simulink model "Wind_DFIG_Reused_R2"  (R2026a)
settings: Solver=ode15s  StopTime=DFIG.Simulation.StopTime  MaxStep=Base.Simulation.MaxStep
InitFcn:
  | root=fileparts(fileparts(get_param(bdroot,'FileName'))); run(fullfile(root,'parameters','init_wind_dfig_reused_r2.m'));
undefined symbols (not defined in the file): Base, Control, Converter, DFIG, Filter, Grid, Wind
libraries: nesl_utility x15, ee_lib x13, fl_lib x5, simulink x1
(part 2 of 2)

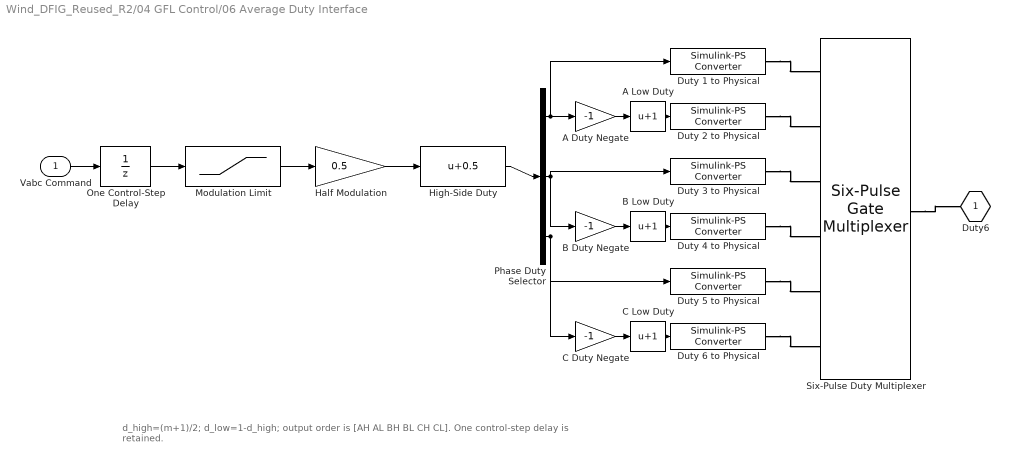
== system Wind_DFIG_Reused_R2/04 GFL Control/06 Average Duty Interface ==
  note: d_high=(m+1)/2; d_low=1-d_high; output order is [AH AL BH BL CH CL]. One control-step delay is retained.
  Vabc Command : Inport
  A Duty Negate : Gain  Gain=-1
  A Low Duty : Bias  Bias=1  SaturateOnIntegerOverflow=off
  B Duty Negate : Gain  Gain=-1
  B Low Duty : Bias  Bias=1  SaturateOnIntegerOverflow=off
  C Duty Negate : Gain  Gain=-1
  C Low Duty : Bias  Bias=1  SaturateOnIntegerOverflow=off
  Duty 1 to Physical : nesl_utility/Simulink-PS Converter  PhysicalDomain=network_engine_domain  SubClassName=ps_input  LeftPortType=input  RightPortType=output  PseudoPeriodic=off  Frequencies=[]  NoiseDistribution=none  NoiseParameters=[]  Unit=V  AffineConversion=off  FilteringAndDerivatives=provide  SimscapeFilterOrder=1  InputFilterTimeConstant=0.001  UdotUserProvided=0
  Duty 2 to Physical : nesl_utility/Simulink-PS Converter  PhysicalDomain=network_engine_domain  SubClassName=ps_input  LeftPortType=input  RightPortType=output  PseudoPeriodic=off  Frequencies=[]  NoiseDistribution=none  NoiseParameters=[]  Unit=V  AffineConversion=off  FilteringAndDerivatives=provide  SimscapeFilterOrder=1  InputFilterTimeConstant=0.001  UdotUserProvided=0
  Duty 3 to Physical : nesl_utility/Simulink-PS Converter  PhysicalDomain=network_engine_domain  SubClassName=ps_input  LeftPortType=input  RightPortType=output  PseudoPeriodic=off  Frequencies=[]  NoiseDistribution=none  NoiseParameters=[]  Unit=V  AffineConversion=off  FilteringAndDerivatives=provide  SimscapeFilterOrder=1  InputFilterTimeConstant=0.001  UdotUserProvided=0
  Duty 4 to Physical : nesl_utility/Simulink-PS Converter  PhysicalDomain=network_engine_domain  SubClassName=ps_input  LeftPortType=input  RightPortType=output  PseudoPeriodic=off  Frequencies=[]  NoiseDistribution=none  NoiseParameters=[]  Unit=V  AffineConversion=off  FilteringAndDerivatives=provide  SimscapeFilterOrder=1  InputFilterTimeConstant=0.001  UdotUserProvided=0
  Duty 5 to Physical : nesl_utility/Simulink-PS Converter  PhysicalDomain=network_engine_domain  SubClassName=ps_input  LeftPortType=input  RightPortType=output  PseudoPeriodic=off  Frequencies=[]  NoiseDistribution=none  NoiseParameters=[]  Unit=V  AffineConversion=off  FilteringAndDerivatives=provide  SimscapeFilterOrder=1  InputFilterTimeConstant=0.001  UdotUserProvided=0
  Duty 6 to Physical : nesl_utility/Simulink-PS Converter  PhysicalDomain=network_engine_domain  SubClassName=ps_input  LeftPortType=input  RightPortType=output  PseudoPeriodic=off  Frequencies=[]  NoiseDistribution=none  NoiseParameters=[]  Unit=V  AffineConversion=off  FilteringAndDerivatives=provide  SimscapeFilterOrder=1  InputFilterTimeConstant=0.001  UdotUserProvided=0
  Half Modulation : Gain  Gain=0.5
  High-Side Duty : Bias  Bias=0.5  SaturateOnIntegerOverflow=off
  Modulation Limit : Saturate  UpperLimit=Converter.ModulationMax  LowerLimit=-Converter.ModulationMax
  One Control-Step Delay : UnitDelay  InitialCondition=[0 0 0]  SampleTime=Control.Ts
  Phase Duty Selector : Demux  Outputs=3
  Six-Pulse Duty Multiplexer : ee_lib/Semiconductors & Converters/Converters/Six-Pulse Gate Multiplexer  port_option=ee.enum.controlport.ps
  Duty6 : PMIOPort  Side=Right
  wires:
  Vabc Command/1 -> One Control-Step Delay/1
  One Control-Step Delay/1 -> Modulation Limit/1
  Modulation Limit/1 -> Half Modulation/1
  Half Modulation/1 -> High-Side Duty/1
  High-Side Duty/1 -> Phase Duty Selector/1
  Phase Duty Selector/1 -> Duty 1 to Physical/1, A Duty Negate/1
  A Duty Negate/1 -> A Low Duty/1
  A Low Duty/1 -> Duty 2 to Physical/1
  Phase Duty Selector/2 -> Duty 3 to Physical/1, B Duty Negate/1
  B Duty Negate/1 -> B Low Duty/1
  B Low Duty/1 -> Duty 4 to Physical/1
  Phase Duty Selector/3 -> Duty 5 to Physical/1, C Duty Negate/1
  C Duty Negate/1 -> C Low Duty/1
  C Low Duty/1 -> Duty 6 to Physical/1
  connections:
  Duty 1 to Physical/RConn1 -- Six-Pulse Duty Multiplexer/LConn1
  Duty 2 to Physical/RConn1 -- Six-Pulse Duty Multiplexer/LConn2
  Duty 3 to Physical/RConn1 -- Six-Pulse Duty Multiplexer/LConn3
  Duty 4 to Physical/RConn1 -- Six-Pulse Duty Multiplexer/LConn4
  Duty 5 to Physical/RConn1 -- Six-Pulse Duty Multiplexer/LConn5
  Duty 6 to Physical/RConn1 -- Six-Pulse Duty Multiplexer/LConn6
  Six-Pulse Duty Multiplexer/RConn1 -- Duty6/RConn1

== system Wind_DFIG_Reused_R2/02 DFIG and Average RSC/02 Wound-Rotor DFIG dq Plant/01 Stator Voltage Equations ==
  Stator Current dq A : Inport
  Stator Flux dq Wb : Inport  Port=2
  Demux Is : Demux  Outputs=2
  Demux Psis : Demux  Outputs=2
  Demux Vs : Demux  Outputs=2
  Mux dPsi_s : Mux  Inputs=2
  Rs ids : Gain  Gain=DFIG.Machine.Rs
  Rs iqs : Gain  Gain=DFIG.Machine.Rs
  Stator Grid Voltage dq : Constant  Value=DFIG.Grid.Vdq
  d_psids_sum : Sum  Inputs=+-+
  d_psiqs_sum : Sum  Inputs=+--
  ws psids : Gain  Gain=DFIG.Base.ws
  ws psiqs : Gain  Gain=DFIG.Base.ws
  dPsi_sdq_dt : Outport
  wires:
  Stator Grid Voltage dq/1 -> Demux Vs/1
  Stator Current dq A/1 -> Demux Is/1
  Stator Flux dq Wb/1 -> Demux Psis/1
  Demux Is/1 -> Rs ids/1
  Demux Is/2 -> Rs iqs/1
  Demux Psis/1 -> ws psids/1
  Demux Psis/2 -> ws psiqs/1
  Demux Vs/1 -> d_psids_sum/1
  Rs ids/1 -> d_psids_sum/2
  ws psiqs/1 -> d_psids_sum/3
  Demux Vs/2 -> d_psiqs_sum/1
  Rs iqs/1 -> d_psiqs_sum/2
  ws psids/1 -> d_psiqs_sum/3
  d_psids_sum/1 -> Mux dPsi_s/1
  d_psiqs_sum/1 -> Mux dPsi_s/2
  Mux dPsi_s/1 -> dPsi_sdq_dt/1

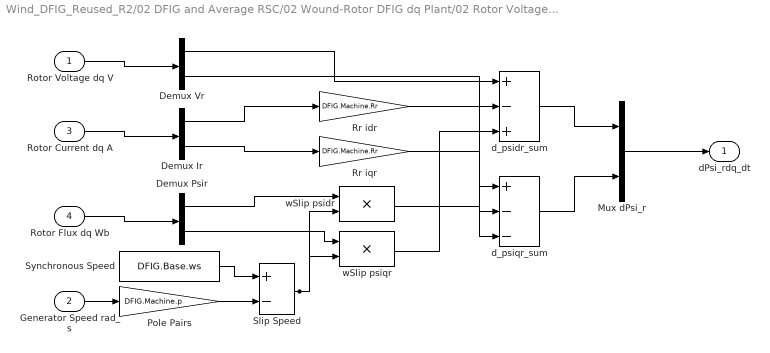
== system Wind_DFIG_Reused_R2/02 DFIG and Average RSC/02 Wound-Rotor DFIG dq Plant/02 Rotor Voltage Equations ==
  Rotor Voltage dq V : Inport
  Generator Speed rad_s : Inport  Port=2
  Rotor Current dq A : Inport  Port=3
  Rotor Flux dq Wb : Inport  Port=4
  Demux Ir : Demux  Outputs=2
  Demux Psir : Demux  Outputs=2
  Demux Vr : Demux  Outputs=2
  Mux dPsi_r : Mux  Inputs=2
  Pole Pairs : Gain  Gain=DFIG.Machine.p
  Rr idr : Gain  Gain=DFIG.Machine.Rr
  Rr iqr : Gain  Gain=DFIG.Machine.Rr
  Slip Speed : Sum  Inputs=+-
  Synchronous Speed : Constant  Value=DFIG.Base.ws
  d_psidr_sum : Sum  Inputs=+-+
  d_psiqr_sum : Sum  Inputs=+--
  wSlip psidr : Product  Inputs=**
  wSlip psiqr : Product  Inputs=**
  dPsi_rdq_dt : Outport
  wires:
  Rotor Voltage dq V/1 -> Demux Vr/1
  Rotor Current dq A/1 -> Demux Ir/1
  Rotor Flux dq Wb/1 -> Demux Psir/1
  Generator Speed rad_s/1 -> Pole Pairs/1
  Synchronous Speed/1 -> Slip Speed/1
  Pole Pairs/1 -> Slip Speed/2
  Demux Ir/1 -> Rr idr/1
  Demux Ir/2 -> Rr iqr/1
  Demux Psir/1 -> wSlip psidr/1
  Slip Speed/1 -> wSlip psidr/2, wSlip psiqr/2
  Demux Psir/2 -> wSlip psiqr/1
  Demux Vr/1 -> d_psidr_sum/1
  Rr idr/1 -> d_psidr_sum/2
  wSlip psiqr/1 -> d_psidr_sum/3
  Demux Vr/2 -> d_psiqr_sum/1
  Rr iqr/1 -> d_psiqr_sum/2
  wSlip psidr/1 -> d_psiqr_sum/3
  d_psidr_sum/1 -> Mux dPsi_r/1
  d_psiqr_sum/1 -> Mux dPsi_r/2
  Mux dPsi_r/1 -> dPsi_rdq_dt/1

== system Wind_DFIG_Reused_R2/02 DFIG and Average RSC/02 Wound-Rotor DFIG dq Plant/03 Flux Integrator and Inductance Matrix ==
  dPsi_sdq_dt : Inport
  dPsi_rdq_dt : Inport  Port=2
  Flux State Integrator : Integrator  InitialCondition=DFIG.Initial.flux
  Flux to Current Matrix : Gain  Gain=DFIG.Machine.CurrentFromFlux  Multiplication=Matrix(K*u)
  Mux State Derivative : Mux  Inputs=2
  Split Stator Rotor Current : Demux  Outputs=[2 2]
  Split Stator Rotor Flux : Demux  Outputs=[2 2]
  Stator Current dq A : Outport
  Rotor Current dq A : Outport  Port=2
  Stator Flux dq Wb : Outport  Port=3
  Rotor Flux dq Wb : Outport  Port=4
  wires:
  dPsi_sdq_dt/1 -> Mux State Derivative/1
  dPsi_rdq_dt/1 -> Mux State Derivative/2
  Mux State Derivative/1 -> Flux State Integrator/1
  Flux State Integrator/1 -> Flux to Current Matrix/1, Split Stator Rotor Flux/1
  Flux to Current Matrix/1 -> Split Stator Rotor Current/1
  Split Stator Rotor Current/1 -> Stator Current dq A/1
  Split Stator Rotor Current/2 -> Rotor Current dq A/1
  Split Stator Rotor Flux/1 -> Stator Flux dq Wb/1
  Split Stator Rotor Flux/2 -> Rotor Flux dq Wb/1

== system Wind_DFIG_Reused_R2/02 DFIG and Average RSC/02 Wound-Rotor DFIG dq Plant/04 Electromagnetic Torque ==
  Stator Current dq A : Inport
  Stator Flux dq Wb : Inport  Port=2
  Air-Gap Flux Cross Product : Sum  Inputs=+-
  Demux Is : Demux  Outputs=2
  Demux Psis : Demux  Outputs=2
  Torque Constant 1.5p : Gain  Gain=1.5*DFIG.Machine.p
  psids iqs : Product  Inputs=**
  psiqs ids : Product  Inputs=**
  Electromagnetic Torque Nm : Outport
  wires:
  Stator Current dq A/1 -> Demux Is/1
  Stator Flux dq Wb/1 -> Demux Psis/1
  Demux Psis/1 -> psids iqs/1
  Demux Is/2 -> psids iqs/2
  Demux Psis/2 -> psiqs ids/1
  Demux Is/1 -> psiqs ids/2
  psids iqs/1 -> Air-Gap Flux Cross Product/1
  psiqs ids/1 -> Air-Gap Flux Cross Product/2
  Air-Gap Flux Cross Product/1 -> Torque Constant 1.5p/1
  Torque Constant 1.5p/1 -> Electromagnetic Torque Nm/1

== system Wind_DFIG_Reused_R2/02 DFIG and Average RSC/03 Rotor-Side Average Converter Control/01 Stator-Flux Current Reference ==
  Torque Reference Nm : Inport
  Idr Magnetizing Reference : Constant  Value=DFIG.RSC.idrRef
  Torque to Iqr Gain : Gain  Gain=DFIG.RSC.torqueToIqr
  Idr_ref_raw_A : Outport
  Iqr_ref_raw_A : Outport  Port=2
  wires:
  Idr Magnetizing Reference/1 -> Idr_ref_raw_A/1
  Torque Reference Nm/1 -> Torque to Iqr Gain/1
  Torque to Iqr Gain/1 -> Iqr_ref_raw_A/1

== system Wind_DFIG_Reused_R2/02 DFIG and Average RSC/03 Rotor-Side Average Converter Control/02 Circular Rotor Current Limiter ==
  Idr_ref_raw_A : Inport
  Iqr_ref_raw_A : Inport  Port=2
  Circular Limit Scale : MinMax  Inputs=2
  Idr Limited : Product  Inputs=**
  Idr Squared : Math  Operator=square
  Iqr Limited : Product  Inputs=**
  Iqr Squared : Math  Operator=square
  Limit Ratio : Product  Inputs=*/
  Magnitude Floor : Constant
  Magnitude Squared : Sum
  Reference Magnitude : Sqrt
  Rotor Current Limit : Constant  Value=DFIG.RSC.Imax
  Safe Magnitude : MinMax  Function=max  Inputs=2
  Unity Scale : Constant
  Idr_ref_lim_A : Outport
  Iqr_ref_lim_A : Outport  Port=2
  wires:
  Idr_ref_raw_A/1 -> Idr Limited/1, Idr Squared/1
  Iqr_ref_raw_A/1 -> Iqr Squared/1, Iqr Limited/2
  Idr Squared/1 -> Magnitude Squared/1
  Iqr Squared/1 -> Magnitude Squared/2
  Magnitude Squared/1 -> Reference Magnitude/1
  Reference Magnitude/1 -> Safe Magnitude/1
  Magnitude Floor/1 -> Safe Magnitude/2
  Rotor Current Limit/1 -> Limit Ratio/1
  Safe Magnitude/1 -> Limit Ratio/2
  Limit Ratio/1 -> Circular Limit Scale/1
  Unity Scale/1 -> Circular Limit Scale/2
  Circular Limit Scale/1 -> Idr Limited/2, Iqr Limited/1
  Idr Limited/1 -> Idr_ref_lim_A/1
  Iqr Limited/1 -> Iqr_ref_lim_A/1

== system Wind_DFIG_Reused_R2/02 DFIG and Average RSC/03 Rotor-Side Average Converter Control/03 Slip and EMF Pre-Control ==
  Rotor Current dq A : Inport
  Generator Speed rad_s : Inport  Port=2
  Rotor Flux dq Wb : Inport  Port=3
  Demux Ir : Demux  Outputs=2
  Demux Psir : Demux  Outputs=2
  Pole Pairs : Gain  Gain=DFIG.Machine.p
  Rr idr : Gain  Gain=DFIG.Machine.Rr
  Rr iqr : Gain  Gain=DFIG.Machine.Rr
  Slip Speed : Sum  Inputs=+-
  Synchronous Speed : Constant  Value=DFIG.Base.ws
  Vdr Pre-Control Sum : Sum  Inputs=+-
  Vqr Pre-Control Sum : Sum
  wSlip psidr : Product  Inputs=**
  wSlip psiqr : Product  Inputs=**
  Vdr_ff_V : Outport
  Vqr_ff_V : Outport  Port=2
  wires:
  Rotor Current dq A/1 -> Demux Ir/1
  Rotor Flux dq Wb/1 -> Demux Psir/1
  Generator Speed rad_s/1 -> Pole Pairs/1
  Synchronous Speed/1 -> Slip Speed/1
  Pole Pairs/1 -> Slip Speed/2
  Demux Ir/1 -> Rr idr/1
  Demux Ir/2 -> Rr iqr/1
  Slip Speed/1 -> wSlip psiqr/1, wSlip psidr/1
  Demux Psir/2 -> wSlip psiqr/2
  Demux Psir/1 -> wSlip psidr/2
  Rr idr/1 -> Vdr Pre-Control Sum/1
  wSlip psiqr/1 -> Vdr Pre-Control Sum/2
  Rr iqr/1 -> Vqr Pre-Control Sum/1
  wSlip psidr/1 -> Vqr Pre-Control Sum/2
  Vdr Pre-Control Sum/1 -> Vdr_ff_V/1
  Vqr Pre-Control Sum/1 -> Vqr_ff_V/1

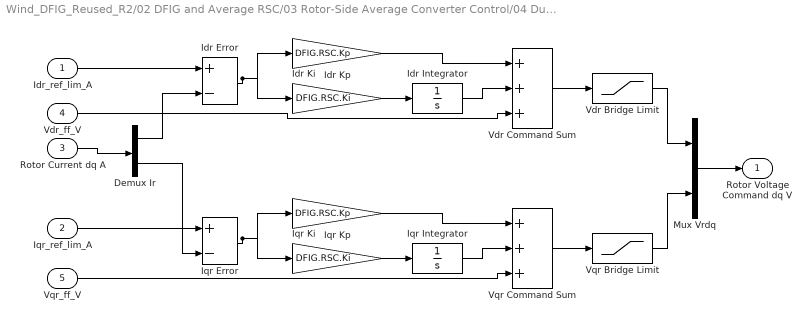
== system Wind_DFIG_Reused_R2/02 DFIG and Average RSC/03 Rotor-Side Average Converter Control/04 Dual-Axis PI and Bridge Limiter ==
  Idr_ref_lim_A : Inport
  Iqr_ref_lim_A : Inport  Port=2
  Rotor Current dq A : Inport  Port=3
  Vdr_ff_V : Inport  Port=4
  Vqr_ff_V : Inport  Port=5
  Demux Ir : Demux  Outputs=2
  Idr Error : Sum  Inputs=+-
  Idr Integrator : Integrator
  Idr Ki : Gain  Gain=DFIG.RSC.Ki
  Idr Kp : Gain  Gain=DFIG.RSC.Kp
  Iqr Error : Sum  Inputs=+-
  Iqr Integrator : Integrator
  Iqr Ki : Gain  Gain=DFIG.RSC.Ki
  Iqr Kp : Gain  Gain=DFIG.RSC.Kp
  Mux Vrdq : Mux  Inputs=2
  Vdr Bridge Limit : Saturate  UpperLimit=DFIG.RSC.Vmax  LowerLimit=-DFIG.RSC.Vmax
  Vdr Command Sum : Sum  Inputs=+++
  Vqr Bridge Limit : Saturate  UpperLimit=DFIG.RSC.Vmax  LowerLimit=-DFIG.RSC.Vmax
  Vqr Command Sum : Sum  Inputs=+++
  Rotor Voltage Command dq V : Outport
  wires:
  Rotor Current dq A/1 -> Demux Ir/1
  Idr_ref_lim_A/1 -> Idr Error/1
  Demux Ir/1 -> Idr Error/2
  Idr Error/1 -> Idr Kp/1, Idr Ki/1
  Idr Ki/1 -> Idr Integrator/1
  Idr Kp/1 -> Vdr Command Sum/1
  Idr Integrator/1 -> Vdr Command Sum/2
  Vdr_ff_V/1 -> Vdr Command Sum/3
  Vdr Command Sum/1 -> Vdr Bridge Limit/1
  Vdr Bridge Limit/1 -> Mux Vrdq/1
  Iqr_ref_lim_A/1 -> Iqr Error/1
  Demux Ir/2 -> Iqr Error/2
  Iqr Error/1 -> Iqr Kp/1, Iqr Ki/1
  Iqr Ki/1 -> Iqr Integrator/1
  Iqr Kp/1 -> Vqr Command Sum/1
  Iqr Integrator/1 -> Vqr Command Sum/2
  Vqr_ff_V/1 -> Vqr Command Sum/3
  Vqr Command Sum/1 -> Vqr Bridge Limit/1
  Vqr Bridge Limit/1 -> Mux Vrdq/2
  Mux Vrdq/1 -> Rotor Voltage Command dq V/1

== system Wind_DFIG_Reused_R2/03 DC Link and Average GSC/Converter AC Measurement/Line Voltage Calculation ==
  Vabc : Inport
  Separate abc : Demux  Outputs=3
  Vab = Va - Vb : Sum  Inputs=+-
  Vab Vbc Vca : Mux  Inputs=3
  Vbc = Vb - Vc : Sum  Inputs=+-
  Vca = Vc - Va : Sum  Inputs=+-
  Vll : Outport
  wires:
  Vabc/1 -> Separate abc/1
  Separate abc/1 -> Vab = Va - Vb/1, Vca = Vc - Va/2
  Separate abc/2 -> Vab = Va - Vb/2, Vbc = Vb - Vc/1
  Separate abc/3 -> Vbc = Vb - Vc/2, Vca = Vc - Va/1
  Vab = Va - Vb/1 -> Vab Vbc Vca/1
  Vbc = Vb - Vc/1 -> Vab Vbc Vca/2
  Vca = Vc - Va/1 -> Vab Vbc Vca/3
  Vab Vbc Vca/1 -> Vll/1  "Vll_inv"

== system Wind_DFIG_Reused_R2/04 GFL Control/01 Measurements and dq/Current alpha beta to dq ==
  alpha beta : Inport
  theta : Inport  Port=2
  Separate alpha beta : Demux  Outputs=2
  alpha cos : Product
  alpha sin : Product
  beta cos : Product
  beta sin : Product
  cos theta : Trigonometry  Operator=cos
  d = alpha cos + beta sin : Sum
  dq vector : Mux  Inputs=2
  q = -alpha sin + beta cos : Sum  Inputs=-+
  sin theta : Trigonometry
  dq : Outport
  wires:
  alpha beta/1 -> Separate alpha beta/1
  theta/1 -> cos theta/1, sin theta/1
  Separate alpha beta/1 -> alpha cos/1, alpha sin/1
  cos theta/1 -> alpha cos/2, beta cos/2
  Separate alpha beta/2 -> beta sin/1, beta cos/1
  sin theta/1 -> beta sin/2, alpha sin/2
  alpha cos/1 -> d = alpha cos + beta sin/1
  beta sin/1 -> d = alpha cos + beta sin/2
  alpha sin/1 -> q = -alpha sin + beta cos/1
  beta cos/1 -> q = -alpha sin + beta cos/2
  d = alpha cos + beta sin/1 -> dq vector/1
  q = -alpha sin + beta cos/1 -> dq vector/2
  dq vector/1 -> dq/1

== system Wind_DFIG_Reused_R2/04 GFL Control/01 Measurements and dq/Voltage alpha beta to dq ==
  alpha beta : Inport
  theta : Inport  Port=2
  Separate alpha beta : Demux  Outputs=2
  alpha cos : Product
  alpha sin : Product
  beta cos : Product
  beta sin : Product
  cos theta : Trigonometry  Operator=cos
  d = alpha cos + beta sin : Sum
  dq vector : Mux  Inputs=2
  q = -alpha sin + beta cos : Sum  Inputs=-+
  sin theta : Trigonometry
  dq : Outport
  wires:
  alpha beta/1 -> Separate alpha beta/1
  theta/1 -> cos theta/1, sin theta/1
  Separate alpha beta/1 -> alpha cos/1, alpha sin/1
  cos theta/1 -> alpha cos/2, beta cos/2
  Separate alpha beta/2 -> beta sin/1, beta cos/1
  sin theta/1 -> beta sin/2, alpha sin/2
  alpha cos/1 -> d = alpha cos + beta sin/1
  beta sin/1 -> d = alpha cos + beta sin/2
  alpha sin/1 -> q = -alpha sin + beta cos/1
  beta cos/1 -> q = -alpha sin + beta cos/2
  d = alpha cos + beta sin/1 -> dq vector/1
  q = -alpha sin + beta cos/1 -> dq vector/2
  dq vector/1 -> dq/1

== system Wind_DFIG_Reused_R2/04 GFL Control/02 Synchronization SRF-PLL/PCC Voltage Prefilter ==
  abc raw : Inport
  Filtered abc : Mux  Inputs=3
  Phase A LPF : TransferFcn  Numerator=[2*pi*Control.PLL.VoltagePrefilterHz]  Denominator=[1 2*pi*Control.PLL.VoltagePrefilterHz]
  Phase B LPF : TransferFcn  Numerator=[2*pi*Control.PLL.VoltagePrefilterHz]  Denominator=[1 2*pi*Control.PLL.VoltagePrefilterHz]
  Phase C LPF : TransferFcn  Numerator=[2*pi*Control.PLL.VoltagePrefilterHz]  Denominator=[1 2*pi*Control.PLL.VoltagePrefilterHz]
  Separate abc : Demux  Outputs=3
  abc filtered : Outport
  wires:
  Separate abc/1 -> Phase A LPF/1
  Phase A LPF/1 -> Filtered abc/1
  Separate abc/2 -> Phase B LPF/1
  Phase B LPF/1 -> Filtered abc/2
  Separate abc/3 -> Phase C LPF/1
  Phase C LPF/1 -> Filtered abc/3
  abc raw/1 -> Separate abc/1
  Filtered abc/1 -> abc filtered/1

== system Wind_DFIG_Reused_R2/04 GFL Control/02 Synchronization SRF-PLL/Park Voltage ==
  alpha beta : Inport
  theta : Inport  Port=2
  Separate alpha beta : Demux  Outputs=2
  alpha cos : Product
  alpha sin : Product
  beta cos : Product
  beta sin : Product
  cos theta : Trigonometry  Operator=cos
  d = alpha cos + beta sin : Sum
  dq vector : Mux  Inputs=2
  q = -alpha sin + beta cos : Sum  Inputs=-+
  sin theta : Trigonometry
  dq : Outport
  wires:
  alpha beta/1 -> Separate alpha beta/1
  theta/1 -> cos theta/1, sin theta/1
  Separate alpha beta/1 -> alpha cos/1, alpha sin/1
  cos theta/1 -> alpha cos/2, beta cos/2
  Separate alpha beta/2 -> beta sin/1, beta cos/1
  sin theta/1 -> beta sin/2, alpha sin/2
  alpha cos/1 -> d = alpha cos + beta sin/1
  beta sin/1 -> d = alpha cos + beta sin/2
  alpha sin/1 -> q = -alpha sin + beta cos/1
  beta cos/1 -> q = -alpha sin + beta cos/2
  d = alpha cos + beta sin/1 -> dq vector/1
  q = -alpha sin + beta cos/1 -> dq vector/2
  dq vector/1 -> dq/1

== system Wind_DFIG_Reused_R2/04 GFL Control/03 DC Voltage and Current Reference/Park Voltage ==
  alpha beta : Inport
  theta : Inport  Port=2
  Separate alpha beta : Demux  Outputs=2
  alpha cos : Product
  alpha sin : Product
  beta cos : Product
  beta sin : Product
  cos theta : Trigonometry  Operator=cos
  d : Sum
  dq vector : Mux  Inputs=2
  q : Sum  Inputs=-+
  sin theta : Trigonometry
  dq : Outport
  wires:
  alpha beta/1 -> Separate alpha beta/1
  theta/1 -> cos theta/1, sin theta/1
  Separate alpha beta/1 -> alpha cos/1, alpha sin/1
  cos theta/1 -> alpha cos/2, beta cos/2
  Separate alpha beta/2 -> beta sin/1, beta cos/1
  sin theta/1 -> beta sin/2, alpha sin/2
  alpha cos/1 -> d/1
  beta sin/1 -> d/2
  alpha sin/1 -> q/1
  beta cos/1 -> q/2
  d/1 -> dq vector/1
  q/1 -> dq vector/2
  dq vector/1 -> dq/1

== system Wind_DFIG_Reused_R2/04 GFL Control/05 dq Current Controller/Inverse Park and Clarke ==
  dq : Inport
  theta : Inport  Port=2
  Inverse Clarke : Gain  Gain=sqrt(2/3)*[1 -0.5 -0.5;0 sqrt(3)/2 -sqrt(3)/2]  Multiplication=Matrix(u*K)
  Separate dq : Demux  Outputs=2
  alpha : Sum  Inputs=+-
  alpha beta : Mux  Inputs=2
  beta : Sum
  cos theta : Trigonometry  Operator=cos
  d cos : Product
  d sin : Product
  q cos : Product
  q sin : Product
  sin theta : Trigonometry
  abc : Outport
  wires:
  dq/1 -> Separate dq/1
  theta/1 -> cos theta/1, sin theta/1
  Separate dq/1 -> d cos/1, d sin/1
  cos theta/1 -> d cos/2, q cos/2
  Separate dq/2 -> q sin/1, q cos/1
  sin theta/1 -> q sin/2, d sin/2
  d cos/1 -> alpha/1
  q sin/1 -> alpha/2
  d sin/1 -> beta/1
  q cos/1 -> beta/2
  alpha/1 -> alpha beta/1
  beta/1 -> alpha beta/2
  alpha beta/1 -> Inverse Clarke/1
  Inverse Clarke/1 -> abc/1

== system Wind_DFIG_Reused_R2/04 GFL Control/05 dq Current Controller/Park Current ==
  alpha beta : Inport
  theta : Inport  Port=2
  Separate alpha beta : Demux  Outputs=2
  alpha cos : Product
  alpha sin : Product
  beta cos : Product
  beta sin : Product
  cos theta : Trigonometry  Operator=cos
  d : Sum
  dq vector : Mux  Inputs=2
  q : Sum  Inputs=-+
  sin theta : Trigonometry
  dq : Outport
  wires:
  alpha beta/1 -> Separate alpha beta/1
  theta/1 -> cos theta/1, sin theta/1
  Separate alpha beta/1 -> alpha cos/1, alpha sin/1
  cos theta/1 -> alpha cos/2, beta cos/2
  Separate alpha beta/2 -> beta sin/1, beta cos/1
  sin theta/1 -> beta sin/2, alpha sin/2
  alpha cos/1 -> d/1
  beta sin/1 -> d/2
  alpha sin/1 -> q/1
  beta cos/1 -> q/2
  d/1 -> dq vector/1
  q/1 -> dq vector/2
  dq vector/1 -> dq/1

== system Wind_DFIG_Reused_R2/04 GFL Control/05 dq Current Controller/Park Voltage ==
  alpha beta : Inport
  theta : Inport  Port=2
  Separate alpha beta : Demux  Outputs=2
  alpha cos : Product
  alpha sin : Product
  beta cos : Product
  beta sin : Product
  cos theta : Trigonometry  Operator=cos
  d : Sum
  dq vector : Mux  Inputs=2
  q : Sum  Inputs=-+
  sin theta : Trigonometry
  dq : Outport
  wires:
  alpha beta/1 -> Separate alpha beta/1
  theta/1 -> cos theta/1, sin theta/1
  Separate alpha beta/1 -> alpha cos/1, alpha sin/1
  cos theta/1 -> alpha cos/2, beta cos/2
  Separate alpha beta/2 -> beta sin/1, beta cos/1
  sin theta/1 -> beta sin/2, alpha sin/2
  alpha cos/1 -> d/1
  beta sin/1 -> d/2
  alpha sin/1 -> q/1
  beta cos/1 -> q/2
  d/1 -> dq vector/1
  q/1 -> dq vector/2
  dq vector/1 -> dq/1
